simulink model "H10_MKC"  (R2026a)
settings: Solver=VariableStepAuto  StopTime=30  MaxStep=2/25
settings Model: Creator=Szalay  LastModifiedBy=Szalay

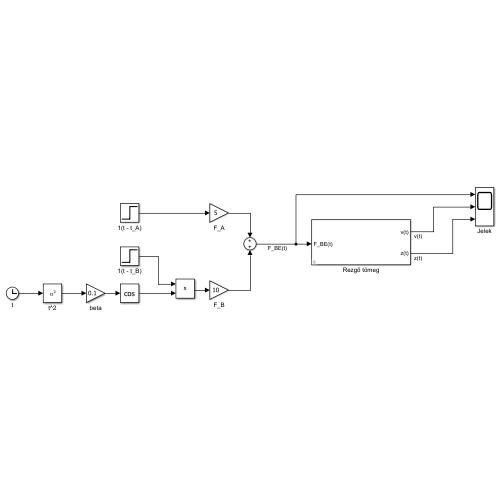
[thumbnail: Simulink's stored preview of the top-level diagram]
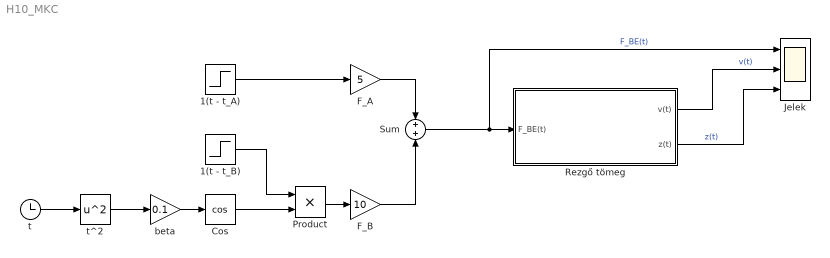
== system H10_MKC ==
  1(t - t_A) : Step  Time=10  SampleTime=0
  1(t - t_B) : Step  Time=20  SampleTime=0
  Cos : Trigonometry  Operator=cos
  F_A : Gain  Gain=5
  F_B : Gain  Gain=10
  Jelek : Scope  NumInputPorts=3
      settings: ActiveDisplayYMinimum=-53.197495279888969  ActiveDisplayYMaximum=22.563537212718025
  Product : Product
  Rezgő tömeg : Subsystem  mask(Rezgő tömeg){m=8, k=4, c=2, z_0=-0.1, v_0=-0.2}
      mask prompts: m "Tömeg"; k "Csillapítási együttható"; c "Rugómerevség"; z_0 "Kezdeti hely"; v_0 "Kezdeti sebesség"
      mask help: Függőleges rezgő tömeg súllyal.
      mask DialogControl ParameterGroupVar Prompt: Modellparaméterek
      mask DialogControl Container3 Prompt: Kezdeti értékek
  Sum : Sum  Inputs=+|+
  beta : Gain  Gain=0.1
  t : Clock
  t^2 : Math  Operator=square
  wires:
  1(t - t_A)/1 -> F_A/1
  Sum/1 -> Jelek/1, Rezgő tömeg/1(F_BE(t))  "F_BE(t)"
  F_A/1 -> Sum/1
  F_B/1 -> Sum/2
  Product/1 -> F_B/1
  1(t - t_B)/1 -> Product/1
  Cos/1 -> Product/2
  beta/1 -> Cos/1
  t/1 -> t^2/1
  t^2/1 -> beta/1
  Rezgő tömeg/1(v(t)) -> Jelek/2  "v(t)"
  Rezgő tömeg/2(z(t)) -> Jelek/3  "z(t)"

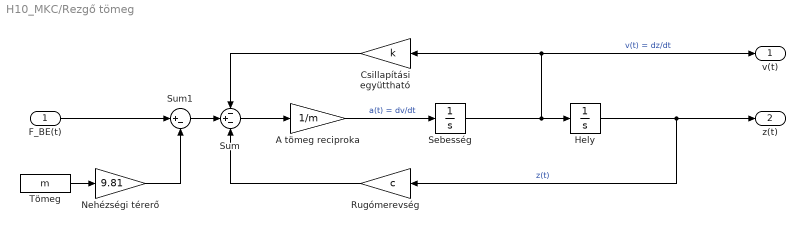
== system H10_MKC/Rezgő tömeg ==
  F_BE(t) : Inport
  A tömeg reciproka : Gain  Gain=1/m
  Csillapítási együttható : Gain  Gain=k
  Hely : Integrator  InitialCondition=z_0
  Nehézségi térerő : Gain  Gain=9.81
  Rugómerevség : Gain  Gain=c
  Sebesség : Integrator  InitialCondition=v_0
  Sum : Sum  Inputs=-+-
  Sum1 : Sum  Inputs=|+-
  Tömeg : Constant  Value=m
  v(t) : Outport
  z(t) : Outport  Port=2
  wires:
  Sebesség/1 -> v(t)/1, Csillapítási együttható/1, Hely/1  "v(t) = dz/dt"
  Hely/1 -> z(t)/1, Rugómerevség/1  "z(t)"
  Sum/1 -> A tömeg reciproka/1
  Csillapítási együttható/1 -> Sum/1
  A tömeg reciproka/1 -> Sebesség/1  "a(t) = dv/dt"
  Sum1/1 -> Sum/2
  F_BE(t)/1 -> Sum1/1
  Tömeg/1 -> Nehézségi térerő/1
  Rugómerevség/1 -> Sum/3
  Nehézségi térerő/1 -> Sum1/2
